simulink subsystem "Shooter_Controls_sub"  (R2023b)
settings: Solver=VariableStepAuto  StartTime=0.0  StopTime=10.0  RelTol=1e-3
undefined symbols (not defined in the file): Feeder_Max_Pulsetime, Field_BlueAllianceZoneX, Field_RedAllianceZoneX, Rebuilt_Feeder_Motor_Gain_FF, Rebuilt_Feeder_Time_FWD, Rebuilt_Feeder_Time_REV, Rebuilt_Hood_Servo_Pos_Min, Rebuilt_Match_Time_Auto_Timer, Rebuilt_Match_Time_End_Game_Timer, Rebuilt_Match_Time_Shift_1, Rebuilt_Match_Time_Shift_2, Rebuilt_Match_Time_Shift_3, Rebuilt_Match_Time_Shift_4, Rebuilt_Match_Time_Shift_Timer, Rebuilt_Match_Time_Shoot_Early, Rebuilt_Match_Time_Transition, Rebuilt_Negative_Feeder_Speed, Rebuilt_Shoot_Hood_Pos_Max_Error, Rebuilt_Shoot_Motor_Max_Error, Rebuilt_Shoot_Robot_Velocity_Max, Rebuilt_Shooter_Error_Integral_Enable, Rebuilt_Shooter_Motor_Gain_FF, Rebuilt_Shooter_Motor_Gain_I, Rebuilt_Shooter_Motor_Gain_I_Low, Rebuilt_Shooter_Motor_Gain_P, Rebuilt_Target_Feeder_Speed, Rebuilt_Target_Transfer_Speed, Rebuilt_Transfer_Error_Integral_Enable, Rebuilt_Transfer_Minimum_Factor, t_sample
libraries: simulink x20, Controls_Components_lib x2
(part 1 of 2)
settings Model: Creator=ander  LastModifiedBy=FIRSTMentor

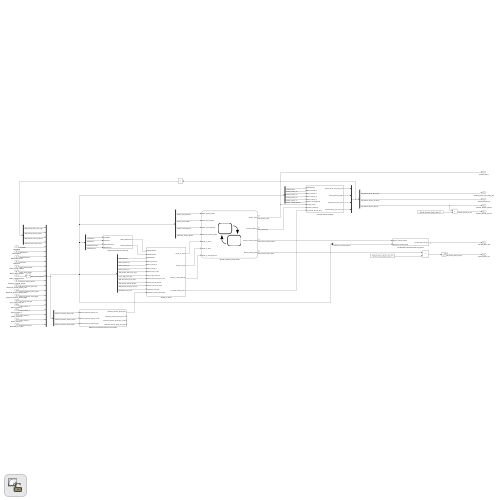
[thumbnail: Simulink's stored preview of the top-level diagram]
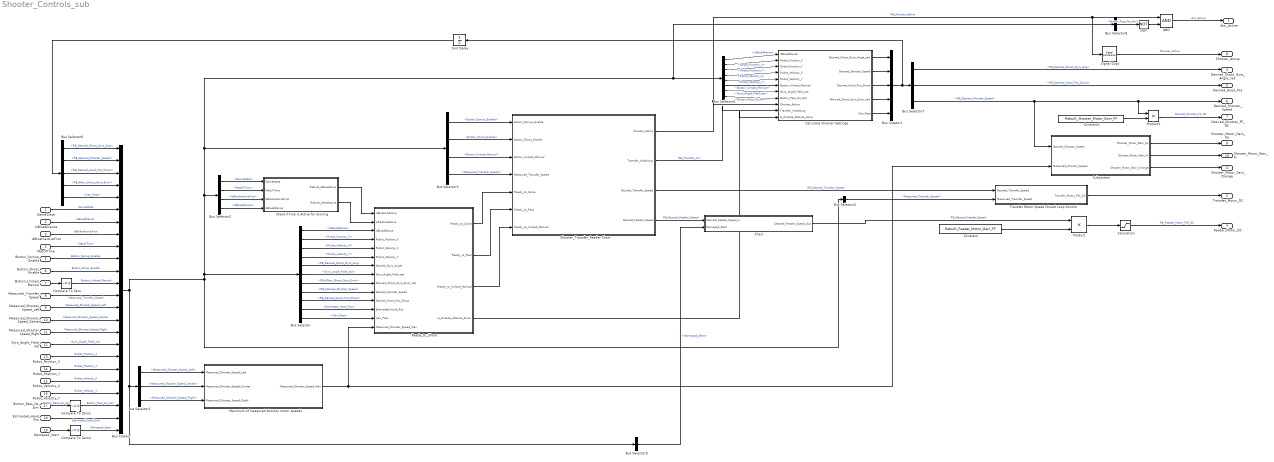
== system Shooter_Controls_sub ==
  GameState : Inport
  IsBlueAlliance : Inport  Port=2
  IsBlueInactiveFirst : Inport  Port=3
  MatchTime : Inport  Port=4
  Button_Spinup_Enable : Inport  Port=5
  Button_Shoot_Enable : Inport  Port=6
  Button_Unload_Manual : Inport  Port=7
  Measured_Transfer_Speed : Inport  Port=8
  Measured_Shooter_Speed_Left : Inport  Port=9
  Measured_Shooter_Speed_Center : Inport  Port=10
  Measured_Shooter_Speed_Right : Inport  Port=11
  Gyro_Angle_Field_rad : Inport  Port=12
  Robot_Position_X : Inport  Port=13
  Robot_Position_Y : Inport  Port=14
  Robot_Velocity_X : Inport  Port=15
  Robot_Velocity_Y : Inport  Port=16
  Button_Pass_No_Aim : Inport  Port=17
  Gamepad_Start : Inport  Port=18
  Estimated_Hood_Pos : Inport  Port=19
  AND : Logic  AllPortsSameDT=off  OutDataTypeStr=boolean
  Bus Creator : BusCreator  Inputs=24
  Bus Selector : BusSelector  OutputSignals=IsBlueAlliance,Robot_Position_X,Robot_Velocity_X,Robot_Velocity_Y,RB_Desired_Shoot_Gyro_Ang,Gyro_Angle_Field_rad,RB_Allow_Shoot_Gyro_Error,RB_Desired_Shooter_Speed,RB_Desired_Hood_Pos_Shoot,Estimated_Hood_Pos,Can_Pass
  Bus Selector1 : BusSelector  OutputSignals=Measured_Shooter_Speed_Left,Measured_Shooter_Speed_Center,Measured_Shooter_Speed_Right
  Bus Selector2 : BusSelector  OutputSignals=GameState,MatchTime,IsBlueInactiveFirst,IsBlueAlliance
  Bus Selector3 : BusSelector  OutputSignals=Button_Spinup_Enable,Button_Shoot_Enable,Button_Unload_Manual,Measured_Transfer_Speed
  Bus Selector4 : BusSelector  OutputSignals=Measured_Transfer_Speed
  Bus Selector5 : BusSelector  OutputSignals=IsBlueAlliance,Robot_Position_X,Robot_Position_Y,Robot_Velocity_X,Robot_Velocity_Y,Button_Unload_Manual,Gyro_Angle_Field_rad,Button_Pass_No_Aim
  Bus Selector6 : BusSelector  OutputSignals=RB_Desired_Shoot_Gyro_Ang,RB_Desired_Shooter_Speed,RB_Desired_Hood_Pos_Shoot,RB_Allow_Shoot_Gyro_Error,Can_Pass
  Bus Selector7 : BusSelector  OutputSignals=RB_Desired_Shoot_Gyro_Ang,RB_Desired_Hood_Pos_Shoot,RB_Desired_Shooter_Speed
  Bus Selector8 : BusSelector  OutputSignals=Button_Pass_No_Aim
  Bus Selector9 : BusSelector  OutputSignals=Gamepad_Start
  Bus Creator1 : BusCreator  Inputs=5
  Calculate Shooter Settings : Subsystem
  Chart : Stateflow chart  TreatAsAtomicUnit=on
  Check if Hub is Active for Scoring : Subsystem
  Compare To Zero : simulink/Logic and Bit Operations/Compare To Zero  relop=~=  OutDataTypeStr=boolean
  Compare To Zero1 : simulink/Logic and Bit Operations/Compare To Zero  relop=~=  OutDataTypeStr=boolean
  Compare To Zero2 : simulink/Logic and Bit Operations/Compare To Zero  relop=~=  OutDataTypeStr=boolean
  Constant : Constant  Value=Rebuilt_Feeder_Motor_Gain_FF
  Constant1 : Constant  Value=Rebuilt_Shooter_Motor_Gain_FF
  Maximum of measured shooter motor speeds : Subsystem
  NOT : Logic  Operator=NOT  AllPortsSameDT=off  OutDataTypeStr=boolean
  Product : Product
  Product1 : Product
  Ready_to_Shoot : Subsystem
  Saturation : Saturate  UpperLimit=1  LowerLimit=-1
  Shooter_Transfer_Feeder Chart : Stateflow chart  TreatAsAtomicUnit=on
      settings: PortSchema="{\"entries\":[{\"content\":{\"sides\":[{\"content\":{\"connectorIds\":[\"In3\",\"In4\",\"In5\",\"In1\",\"In2\",\"In6\",\"In7\"]},\"type\":\"ConnectorPlacement.EquallySpacedRectSide\",\"uuid\":\"74f441ca-e68c-42da-ab23-bb4c7b61ec4f\"},{\"content\":{\"connectorIds\":[\"Out1\",\"Out4\",\"Out3\",\"Out2\"],\"side\":\"RIGHT\"},\"type\":\"ConnectorPlacement.EquallySpacedRectSide\",\"uuid\":\"2fadc481-2bc8-4130-a1bd-49ae230fca41\"},{\"content\":{\"side\":\"TOP\"},\"type\":\"ConnectorPlacement.EquallySpacedRectSide\",\"uuid\":\"2ae77c41-2153-497e-bbb0-d4cfaeee089b\"}]},\"type\":\"ConnectorPlacement.EquallySpacedConnector\",\"uuid\":\"7b036f05-bc25-4046-a317-cc0a6fa71ced\"}],\"packageUris\":[\"http://schema.mathworks.com/mf0/Connector/R2020b\"],\"version\":\"1.0\"}"
  Signal Copy : SignalConversion  OverrideOpt=off
  Subsystem : Subsystem
  Transfer Motor Speed Closed Loop Control : Subsystem
  Unit Delay : UnitDelay  SampleTime=-1  HasFrameUpgradeWarning=on
  Aim_Active : Outport
  Transfer_Motor_DC : Outport  Port=2
  Feeder_Motor_DC : Outport  Port=3
  Desired_Shoot_Gyro_Angle_rad : Outport  Port=4
  Desired_Hood_Pos : Outport  Port=5
  Desired_Shooter_Speed : Outport  Port=6
  Desired_Shooter_FF_DC : Outport  Port=7
  Shooter_Active : Outport  Port=8
  Shooter_Motor_Gain_Kp : Outport  Port=9
  Shooter_Motor_Gain_Ki : Outport  Port=10
  Shooter_Motor_Gain_Change : Outport  Port=11
  wires:
  Shooter_Transfer_Feeder Chart/1(Shooter_Active) -> Calculate Shooter Settings/9(Shooter_Active), Signal Copy/1, AND/1  "RB_Shooter_Active"
  Check if Hub is Active for Scoring/1(Rebuilt_IsBlueActive) -> Ready_to_Shoot/1(isBlueHubActive)
  Check if Hub is Active for Scoring/2(Rebuilt_IsRedActive) -> Ready_to_Shoot/2(isRedHubActive)
  Ready_to_Shoot/1(Ready_to_Score) -> Shooter_Transfer_Feeder Chart/2(Ready_to_Score)
  Bus Creator/1 -> Bus Selector1/1, Bus Selector9/1, Bus Selector4/1, Bus Selector2/1, Bus Selector3/1, Bus Selector5/1, Bus Selector8/1, Bus Selector/1
  Bus Selector/6 -> Ready_to_Shoot/8(Gyro_Angle_Field_rad)  "<Gyro_Angle_Field_rad>"
  Bus Selector/5 -> Ready_to_Shoot/7(Desired_Gyro_Angle)  "<RB_Desired_Shoot_Gyro_Ang>"
  Bus Selector/8 -> Ready_to_Shoot/10(Desired_Shooter_Speed)  "<RB_Desired_Shooter_Speed>"
  Bus Selector/2 -> Ready_to_Shoot/4(Robot_Position_X)  "<Robot_Position_X>"
  Bus Selector/1 -> Ready_to_Shoot/3(isBlueAlliance)  "<IsBlueAlliance>"
  Bus Selector2/2 -> Check if Hub is Active for Scoring/2(MatchTime)  "<MatchTime>"
  Bus Selector2/3 -> Check if Hub is Active for Scoring/3(IsBlueInactiveFirst)  "<IsBlueInactiveFirst>"
  Bus Selector3/1 -> Shooter_Transfer_Feeder Chart/3(Button_Spinup_Enable)  "<Button_Spinup_Enable>"
  Bus Selector3/2 -> Shooter_Transfer_Feeder Chart/4(Button_Shoot_Enable)  "<Button_Shoot_Enable>"
  Bus Selector3/4 -> Shooter_Transfer_Feeder Chart/1(Measured_Transfer_Speed)  "<Measured_Transfer_Speed>"
  Product/1 -> Saturation/1
  Shooter_Transfer_Feeder Chart/3(Desired_Transfer_Speed) -> Transfer Motor Speed Closed Loop Control/1(Desired_Transfer_Speed)  "RB_Desired_Transfer_Speed"
  Bus Selector4/1 -> Transfer Motor Speed Closed Loop Control/2(Measured_Transfer_Speed)  "<Measured_Transfer_Speed>"
  Transfer Motor Speed Closed Loop Control/1(Transfer_Motor_PID_DC) -> Transfer_Motor_DC/1
  Bus Selector5/2 -> Calculate Shooter Settings/2(Robot_Position_X)  "<Robot_Position_X>"
  Bus Selector5/3 -> Calculate Shooter Settings/3(Robot_Position_Y)  "<Robot_Position_Y>"
  Calculate Shooter Settings/1(Desired_Shoot_Gyro_Angle_rad) -> Bus Creator1/1
  Calculate Shooter Settings/2(Desired_Shooter_Speed) -> Bus Creator1/2
  Calculate Shooter Settings/3(Desired_Hood_Pos_Shoot) -> Bus Creator1/3
  Bus Creator1/1 -> Bus Selector7/1, Unit Delay/1
  Unit Delay/1 -> Bus Selector6/1
  Bus Selector5/1 -> Calculate Shooter Settings/1(IsBlueAlliance)  "<IsBlueAlliance>"
  Constant/1 -> Product/2
  Bus Selector6/1 -> Bus Creator/1  "<RB_Desired_Shoot_Gyro_Ang>"
  Bus Selector6/2 -> Bus Creator/2  "<RB_Desired_Shooter_Speed>"
  Bus Selector6/3 -> Bus Creator/3  "<RB_Desired_Hood_Pos_Shoot>"
  Gyro_Angle_Field_rad/1 -> Bus Creator/17  "Gyro_Angle_Field_rad"
  Robot_Position_X/1 -> Bus Creator/18  "Robot_Position_X"
  Robot_Position_Y/1 -> Bus Creator/19  "Robot_Position_Y"
  Robot_Velocity_X/1 -> Bus Creator/20  "Robot_Velocity_X"
  Robot_Velocity_Y/1 -> Bus Creator/21  "Robot_Velocity_Y"
  Bus Selector5/4 -> Calculate Shooter Settings/4(Robot_Velocity_X)  "<Robot_Velocity_X>"
  Bus Selector5/5 -> Calculate Shooter Settings/5(Robot_Velocity_Y)  "<Robot_Velocity_Y>"
  Bus Selector7/1 -> Desired_Shoot_Gyro_Angle_rad/1  "<RB_Desired_Shoot_Gyro_Ang>"
  Bus Selector7/2 -> Desired_Hood_Pos/1  "<RB_Desired_Hood_Pos_Shoot>"
  Bus Selector7/3 -> Desired_Shooter_Speed/1, Product1/1, Subsystem/1(Desired_Shooter_Speed)  "<RB_Desired_Shooter_Speed>"
  Ready_to_Shoot/2(Ready_to_Pass) -> Shooter_Transfer_Feeder Chart/6(Ready_to_Pass)
  Ready_to_Shoot/4(Is_Outside_Alliance_Zone) -> Calculate Shooter Settings/11(Is_Outside_Alliance_Zone)
  Bus Selector2/1 -> Check if Hub is Active for Scoring/1(GameState)  "<GameState>"
  GameState/1 -> Bus Creator/6  "GameState"
  IsBlueAlliance/1 -> Bus Creator/7  "IsBlueAlliance"
  IsBlueInactiveFirst/1 -> Bus Creator/8  "IsBlueInactiveFirst"
  MatchTime/1 -> Bus Creator/9  "MatchTime"
  Button_Spinup_Enable/1 -> Bus Creator/10  "Button_Spinup_Enable"
  Button_Shoot_Enable/1 -> Bus Creator/11  "Button_Shoot_Enable"
  Measured_Transfer_Speed/1 -> Bus Creator/13  "Measured_Transfer_Speed"
  Measured_Shooter_Speed_Left/1 -> Bus Creator/14  "Measured_Shooter_Speed_Left"
  Measured_Shooter_Speed_Center/1 -> Bus Creator/15  "Measured_Shooter_Speed_Center"
  Measured_Shooter_Speed_Right/1 -> Bus Creator/16  "Measured_Shooter_Speed_Right"
  Calculate Shooter Settings/4(Allowed_Shoot_Gyro_Error_rad) -> Bus Creator1/4
  Bus Selector6/4 -> Bus Creator/4  "<RB_Allow_Shoot_Gyro_Error>"
  Bus Selector/3 -> Ready_to_Shoot/5(Robot_Velocity_X)  "<Robot_Velocity_X>"
  Bus Selector/4 -> Ready_to_Shoot/6(Robot_Velocity_Y)  "<Robot_Velocity_Y>"
  Bus Selector/7 -> Ready_to_Shoot/9(Allowed_Shoot_Gyro_Error_rad)  "<RB_Allow_Shoot_Gyro_Error>"
  Bus Selector/9 -> Ready_to_Shoot/11(Desired_Hood_Pos_Shoot)  "<RB_Desired_Hood_Pos_Shoot>"
  Bus Selector1/1 -> Maximum of measured shooter motor speeds/1(Measured_Shooter_Speed_Left)  "<Measured_Shooter_Speed_Left>"
  Bus Selector1/2 -> Maximum of measured shooter motor speeds/2(Measured_Shooter_Speed_Center)  "<Measured_Shooter_Speed_Center>"
  Bus Selector1/3 -> Maximum of measured shooter motor speeds/3(Measured_Shooter_Speed_Right)  "<Measured_Shooter_Speed_Right>"
  Bus Selector/10 -> Ready_to_Shoot/12(Estimated_Hood_Pos)  "<Estimated_Hood_Pos>"
  Shooter_Transfer_Feeder Chart/4(Transfer_Initializing) -> Calculate Shooter Settings/10(Transfer_Initializing)  "RB_Transfer_Init"
  Saturation/1 -> Feeder_Motor_DC/1  "RB_Feeder_Motor_PID_DC"
  Bus Selector2/4 -> Check if Hub is Active for Scoring/4(IsBlueAlliance)  "<IsBlueAlliance>"
  Ready_to_Shoot/3(Ready_to_Unload_Manual) -> Shooter_Transfer_Feeder Chart/7(Ready_to_Unload_Manual)
  Button_Unload_Manual/1 -> Compare To Zero/1
  Bus Selector3/3 -> Shooter_Transfer_Feeder Chart/5(Button_Unload_Manual)  "<Button_Unload_Manual>"
  Bus Selector5/6 -> Calculate Shooter Settings/6(Button_Unload_Manual)  "<Button_Unload_Manual>"
  Compare To Zero/1 -> Bus Creator/12  "Button_Unload_Manual"
  Product1/1 -> Desired_Shooter_FF_DC/1  "Desired_Shooter_FF_DC"
  Constant1/1 -> Product1/2
  Bus Selector5/7 -> Calculate Shooter Settings/7(Gyro_Angle_Field_rad)  "<Gyro_Angle_Field_rad>"
  Bus Selector5/8 -> Calculate Shooter Settings/8(Button_Pass_No_Aim)  "<Button_Pass_No_Aim>"
  AND/1 -> Aim_Active/1  "Aim_Active"
  Calculate Shooter Settings/5(Can_Pass) -> Bus Creator1/5
  Bus Selector8/1 -> NOT/1  "<Button_Pass_No_Aim>"
  Signal Copy/1 -> Shooter_Active/1  "Shooter_Active"
  Bus Selector6/5 -> Bus Creator/5  "<Can_Pass>"
  Estimated_Hood_Pos/1 -> Bus Creator/23  "Estimated_Hood_Pos"
  Button_Pass_No_Aim/1 -> Compare To Zero1/1  "Button_Pass_No_Aim"
  Bus Selector/11 -> Ready_to_Shoot/13(Can_Pass)  "<Can_Pass>"
  NOT/1 -> AND/2
  Compare To Zero1/1 -> Bus Creator/22  "Button_Pass_No_Aim"
  Maximum of measured shooter motor speeds/1(Measured_Shooter_Speed_Max) -> Ready_to_Shoot/14(Measured_Shooter_Speed_Max), Subsystem/2(Measured_Shooter_Speed)
  Subsystem/1(Shooter_Motor_Gain_Kp) -> Shooter_Motor_Gain_Kp/1
  Subsystem/2(Shooter_Motor_Gain_Ki) -> Shooter_Motor_Gain_Ki/1
  Subsystem/3(Shooter_Motor_Gain_Change) -> Shooter_Motor_Gain_Change/1
  Gamepad_Start/1 -> Compare To Zero2/1
  Bus Selector9/1 -> Chart/2(Gamepad_Start)  "<Gamepad_Start>"
  Shooter_Transfer_Feeder Chart/2(Desired_Feeder_Speed) -> Chart/1(Desired_Feeder_Speed_In)  "RB_Desired_Feeder_Speed"
  Chart/1(Desired_Feeder_Speed_Out) -> Product/1  "RB_Desired_Feeder_Speed"
  Compare To Zero2/1 -> Bus Creator/24  "Gamepad_Start"

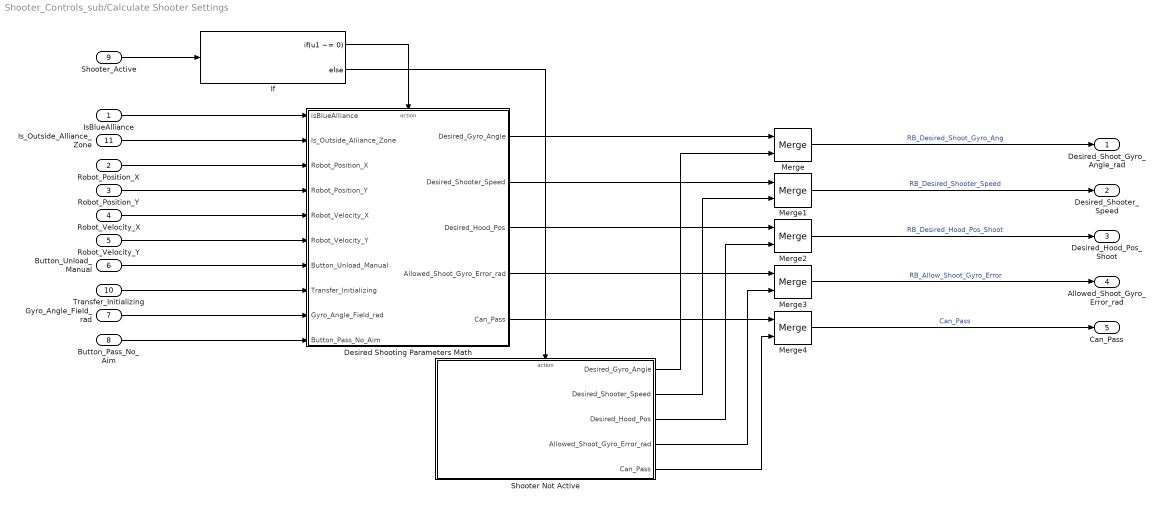
== system Shooter_Controls_sub/Calculate Shooter Settings ==
  IsBlueAlliance : Inport
  Robot_Position_X : Inport  Port=2
  Robot_Position_Y : Inport  Port=3
  Robot_Velocity_X : Inport  Port=4
  Robot_Velocity_Y : Inport  Port=5
  Button_Unload_Manual : Inport  Port=6
  Gyro_Angle_Field_rad : Inport  Port=7
  Button_Pass_No_Aim : Inport  Port=8
  Shooter_Active : Inport  Port=9
  Transfer_Initializing : Inport  Port=10
  Is_Outside_Alliance_Zone : Inport  Port=11
  Desired Shooting Parameters Math : Subsystem
  If : If  IfExpression=u1 ~= 0
  Merge{,1..4} (5 alike) : Merge
  Shooter Not Active : Subsystem
  Desired_Shoot_Gyro_Angle_rad : Outport
  Desired_Shooter_Speed : Outport  Port=2
  Desired_Hood_Pos_Shoot : Outport  Port=3
  Allowed_Shoot_Gyro_Error_rad : Outport  Port=4
  Can_Pass : Outport  Port=5
  wires:
  Merge4/1 -> Can_Pass/1  "Can_Pass"
  Shooter Not Active/5(Can_Pass) -> Merge4/2
  Desired Shooting Parameters Math/5(Can_Pass) -> Merge4/1
  Button_Pass_No_Aim/1 -> Desired Shooting Parameters Math/10(Button_Pass_No_Aim)
  Gyro_Angle_Field_rad/1 -> Desired Shooting Parameters Math/9(Gyro_Angle_Field_rad)
  Button_Unload_Manual/1 -> Desired Shooting Parameters Math/7(Button_Unload_Manual)
  Transfer_Initializing/1 -> Desired Shooting Parameters Math/8(Transfer_Initializing)
  Is_Outside_Alliance_Zone/1 -> Desired Shooting Parameters Math/2(Is_Outside_Alliance_Zone)
  Shooter Not Active/4(Allowed_Shoot_Gyro_Error_rad) -> Merge3/2
  Shooter Not Active/3(Desired_Hood_Pos) -> Merge2/2
  Shooter Not Active/2(Desired_Shooter_Speed) -> Merge1/2
  Shooter Not Active/1(Desired_Gyro_Angle) -> Merge/2
  Desired Shooting Parameters Math/4(Allowed_Shoot_Gyro_Error_rad) -> Merge3/1
  Desired Shooting Parameters Math/3(Desired_Hood_Pos) -> Merge2/1
  Desired Shooting Parameters Math/2(Desired_Shooter_Speed) -> Merge1/1
  Desired Shooting Parameters Math/1(Desired_Gyro_Angle) -> Merge/1
  Robot_Velocity_Y/1 -> Desired Shooting Parameters Math/6(Robot_Velocity_Y)
  Robot_Velocity_X/1 -> Desired Shooting Parameters Math/5(Robot_Velocity_X)
  Robot_Position_Y/1 -> Desired Shooting Parameters Math/4(Robot_Position_Y)
  Robot_Position_X/1 -> Desired Shooting Parameters Math/3(Robot_Position_X)
  IsBlueAlliance/1 -> Desired Shooting Parameters Math/1(isBlueAlliance)
  Merge3/1 -> Allowed_Shoot_Gyro_Error_rad/1  "RB_Allow_Shoot_Gyro_Error"
  If/2 -> Shooter Not Active/Action
  Shooter_Active/1 -> If/1
  Merge1/1 -> Desired_Shooter_Speed/1  "RB_Desired_Shooter_Speed"
  If/1 -> Desired Shooting Parameters Math/Action
  Merge/1 -> Desired_Shoot_Gyro_Angle_rad/1  "RB_Desired_Shoot_Gyro_Ang"
  Merge2/1 -> Desired_Hood_Pos_Shoot/1  "RB_Desired_Hood_Pos_Shoot"

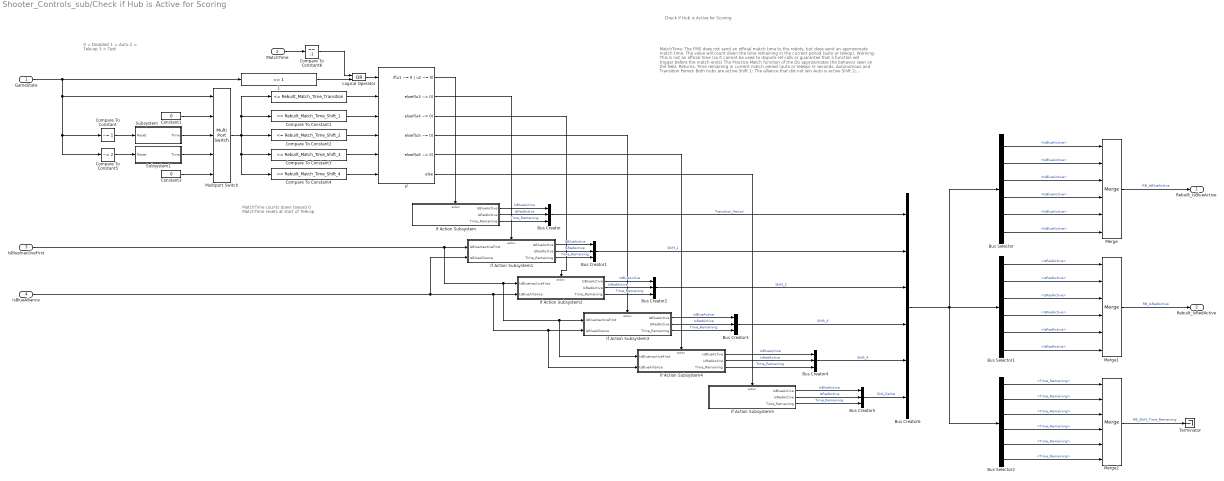
== system Shooter_Controls_sub/Check if Hub is Active for Scoring ==
  note: MatchTime counts down toward 0
      | MatchTime resets at start of Tele-op
  note: Check if Hub is Active for Scoring
  note: MatchTime: The FMS does not send an official match time to the robots, but does send an approximate match time. The value will count down the time remaining in the current period (auto or teleop). Warning: This is not an official time (so it cannot be used to dispute ref calls or guarantee that a function will trigger before the match ends) The Practice Match function of the DS approximates the behavior seen on the field.
      | Returns: Time remaining in current match period (auto or teleop) in seconds.
      |
      | Autonomous and Transition Period: Both hubs are active
      | Shift 1: The alliance that did not win Auto is active
      | Shift 2: Opposite of Shift 1
      | Shift 3: Same as Shift 1
      | Shift 4: Same as Shift 2
      | Endgame: Both hubs are active
  note: 0 = Disabled
      | 1 = Auto
      | 2 = Tele-op
      | 3 = Test
  GameState : Inport
  MatchTime : Inport  Port=2
  IsBlueInactiveFirst : Inport  Port=3
  IsBlueAlliance : Inport  Port=4
  " " : simulink/Logic and Bit Operations/Compare To Constant  relop=<=  const=Rebuilt_Match_Time_Transition  OutDataTypeStr=boolean
  " 1" : simulink/Logic and Bit Operations/Compare To Constant  relop===  const=1  OutDataTypeStr=boolean
  Bus Creator{,1..5} (6 alike) : BusCreator  Inputs=3
  Bus Creator6 : BusCreator  Inputs=6
  Bus Selector : BusSelector  OutputSignals=Transition_Period.IsBlueActive,Shift_1.IsBlueActive,Shift_2.IsBlueActive,Shift_3.IsBlueActive,Shift_4.IsBlueActive,End_Game.IsBlueActive
  Bus Selector1 : BusSelector  OutputSignals=Transition_Period.IsRedActive,Shift_1.IsRedActive,Shift_2.IsRedActive,Shift_3.IsRedActive,Shift_4.IsRedActive,End_Game.IsRedActive
  Bus Selector2 : BusSelector  OutputSignals=Transition_Period.Time_Remaining,Shift_1.Time_Remaining,Shift_2.Time_Remaining,Shift_3.Time_Remaining,Shift_4.Time_Remaining,End_Game.Time_Remaining
  Compare To Constant : simulink/Logic and Bit Operations/Compare To Constant  relop=~=  const=1  OutDataTypeStr=boolean
  Compare To Constant1 : simulink/Logic and Bit Operations/Compare To Constant  relop=<=  const=Rebuilt_Match_Time_Shift_1  OutDataTypeStr=boolean
  Compare To Constant2 : simulink/Logic and Bit Operations/Compare To Constant  relop=<=  const=Rebuilt_Match_Time_Shift_2  OutDataTypeStr=boolean
  Compare To Constant3 : simulink/Logic and Bit Operations/Compare To Constant  relop=<=  const=Rebuilt_Match_Time_Shift_3  OutDataTypeStr=boolean
  Compare To Constant4 : simulink/Logic and Bit Operations/Compare To Constant  relop=<=  const=Rebuilt_Match_Time_Shift_4  OutDataTypeStr=boolean
  Compare To Constant5 : simulink/Logic and Bit Operations/Compare To Constant  relop=~=  const=2  OutDataTypeStr=boolean
  Compare To Constant6 : simulink/Logic and Bit Operations/Compare To Constant  relop===  const=-1  OutDataTypeStr=boolean
  Constant1 : Constant  Value=0
  Constant3 : Constant  Value=0
  If : If  NumInputs=6  IfExpression=u1 ~= 0 | u2 ~= 0  ElseIfExpressions=u3 ~= 0,u4 ~= 0,u5 ~= 0,u6 ~= 0
  If Action Subsystem : Subsystem  TreatAsAtomicUnit=on
  If Action Subsystem1 : Subsystem  TreatAsAtomicUnit=on
  If Action Subsystem2 : Subsystem  TreatAsAtomicUnit=on
  If Action Subsystem3 : Subsystem  TreatAsAtomicUnit=on
  If Action Subsystem4 : Subsystem  TreatAsAtomicUnit=on
  If Action Subsystem5 : Subsystem  TreatAsAtomicUnit=on
  Logical Operator : Logic  Operator=OR  AllPortsSameDT=off  OutDataTypeStr=boolean
  Merge : Merge  Inputs=6
  Merge1 : Merge  Inputs=6
  Merge2 : Merge  Inputs=6
  Multiport Switch : MultiPortSwitch  DataPortOrder=Zero-based contiguous  Inputs=4  zeroidx=on  SaturateOnIntegerOverflow=off  InputSameDT=off
  Subsystem : Subsystem
  Subsystem1 : Subsystem
  Terminator : Terminator
  Rebuilt_IsBlueActive : Outport
  Rebuilt_IsRedActive : Outport  Port=2
  wires:
  Compare To Constant6/1 -> Logical Operator/1
  Logical Operator/1 -> If/1
  " 1"/1 -> Logical Operator/2
  MatchTime/1 -> Compare To Constant6/1
  Compare To Constant5/1 -> Subsystem1/1(Reset)
  Subsystem1/1(Time) -> Multiport Switch/4
  Compare To Constant/1 -> Subsystem/1(Reset)
  Subsystem/1(Time) -> Multiport Switch/3
  Constant3/1 -> Multiport Switch/5
  Constant1/1 -> Multiport Switch/2
  Multiport Switch/1 -> " "/1, Compare To Constant1/1, Compare To Constant4/1, Compare To Constant3/1, Compare To Constant2/1
  IsBlueAlliance/1 -> If Action Subsystem2/2(IsBlueAlliance), If Action Subsystem3/2(IsBlueAlliance), If Action Subsystem4/2(IsBlueAlliance), If Action Subsystem1/2(IsBlueAlliance)
  GameState/1 -> Multiport Switch/1, Compare To Constant/1, Compare To Constant5/1, " 1"/1
  Compare To Constant4/1 -> If/6
  Compare To Constant3/1 -> If/5
  Compare To Constant2/1 -> If/4
  Compare To Constant1/1 -> If/3
  " "/1 -> If/2
  If Action Subsystem5/3(Time_Remaining) -> Bus Creator5/3  "Time_Remaining"
  If Action Subsystem4/3(Time_Remaining) -> Bus Creator4/3  "Time_Remaining"
  If Action Subsystem3/3(Time_Remaining) -> Bus Creator3/3  "Time_Remaining"
  If Action Subsystem2/3(Time_Remaining) -> Bus Creator2/3  "Time_Remaining"
  Merge2/1 -> Terminator/1  "RB_Shift_Time_Remaining"
  Bus Selector2/6 -> Merge2/6  "<Time_Remaining>"
  Bus Selector2/5 -> Merge2/5  "<Time_Remaining>"
  Bus Selector2/4 -> Merge2/4  "<Time_Remaining>"
  Bus Selector2/3 -> Merge2/3  "<Time_Remaining>"
  Bus Selector2/2 -> Merge2/2  "<Time_Remaining>"
  Bus Selector2/1 -> Merge2/1  "<Time_Remaining>"
  Bus Selector1/6 -> Merge1/6  "<IsRedActive>"
  Bus Selector1/5 -> Merge1/5  "<IsRedActive>"
  Bus Selector1/4 -> Merge1/4  "<IsRedActive>"
  Bus Selector1/3 -> Merge1/3  "<IsRedActive>"
  Bus Selector1/2 -> Merge1/2  "<IsRedActive>"
  Bus Selector1/1 -> Merge1/1  "<IsRedActive>"
  Bus Selector/6 -> Merge/6  "<IsBlueActive>"
  Bus Selector/5 -> Merge/5  "<IsBlueActive>"
  Bus Selector/4 -> Merge/4  "<IsBlueActive>"
  Bus Selector/3 -> Merge/3  "<IsBlueActive>"
  Bus Selector/2 -> Merge/2  "<IsBlueActive>"
  Bus Selector/1 -> Merge/1  "<IsBlueActive>"
  Bus Creator6/1 -> Bus Selector2/1, Bus Selector1/1, Bus Selector/1
  Bus Creator5/1 -> Bus Creator6/6  "End_Game"
  Bus Creator4/1 -> Bus Creator6/5  "Shift_4"
  Bus Creator3/1 -> Bus Creator6/4  "Shift_3"
  Bus Creator2/1 -> Bus Creator6/3  "Shift_2"
  Bus Creator1/1 -> Bus Creator6/2  "Shift_1"
  Bus Creator/1 -> Bus Creator6/1  "Transition_Period"
  If Action Subsystem5/2(IsRedActive) -> Bus Creator5/2  "IsRedActive"
  If Action Subsystem5/1(IsBlueActive) -> Bus Creator5/1  "IsBlueActive"
  If Action Subsystem4/2(IsRedActive) -> Bus Creator4/2  "IsRedActive"
  If Action Subsystem4/1(IsBlueActive) -> Bus Creator4/1  "IsBlueActive"
  If Action Subsystem3/2(IsRedActive) -> Bus Creator3/2  "IsRedActive"
  If Action Subsystem3/1(IsBlueActive) -> Bus Creator3/1  "IsBlueActive"
  If Action Subsystem2/2(IsRedActive) -> Bus Creator2/2  "IsRedActive"
  If Action Subsystem2/1(IsBlueActive) -> Bus Creator2/1  "IsBlueActive"
  If Action Subsystem1/3(Time_Remaining) -> Bus Creator1/3  "Time_Remaining"
  If Action Subsystem1/2(IsRedActive) -> Bus Creator1/2  "IsRedActive"
  If Action Subsystem1/1(IsBlueActive) -> Bus Creator1/1  "IsBlueActive"
  If Action Subsystem/3(Time_Remaining) -> Bus Creator/3  "Time_Remaining"
  If Action Subsystem/2(IsRedActive) -> Bus Creator/2  "IsRedActive"
  If Action Subsystem/1(IsBlueActive) -> Bus Creator/1  "IsBlueActive"
  Merge1/1 -> Rebuilt_IsRedActive/1  "RB_IsRedActive"
  Merge/1 -> Rebuilt_IsBlueActive/1  "RB_IsBlueActive"
  If/6 -> If Action Subsystem5/Action
  If/5 -> If Action Subsystem4/Action
  If/4 -> If Action Subsystem3/Action
  If/3 -> If Action Subsystem2/Action
  If/2 -> If Action Subsystem1/Action
  IsBlueInactiveFirst/1 -> If Action Subsystem1/1(IsBlueInactiveFirst), If Action Subsystem2/1(IsBlueInactiveFirst), If Action Subsystem3/1(IsBlueInactiveFirst), If Action Subsystem4/1(IsBlueInactiveFirst)
  If/1 -> If Action Subsystem/Action

== system Shooter_Controls_sub/Maximum of measured shooter motor speeds ==
  note: The three sets of shooter wheels are all connected together on a single hex shaft.
      |
      | Three motors are connected to the single hex shaft through independent belts and pulleys.
      |
      | Each of the motors are running close to the same speed, but not exactly due to the slight differences in pulleys and flex in the belts.
      |
      | Take the absolute value of each motor speed (mounting differences will cause some to be positive and others negative) and then take the maximum of the three. This allows the robot to keep working if one motor fails.
  note: Calculate Measured Shooter Motor Speed Maximum
  Measured_Shooter_Speed_Left : Inport
  Measured_Shooter_Speed_Center : Inport  Port=2
  Measured_Shooter_Speed_Right : Inport  Port=3
  Abs1 : Abs  SaturateOnIntegerOverflow=off
  Abs2 : Abs  SaturateOnIntegerOverflow=off
  Abs3 : Abs  SaturateOnIntegerOverflow=off
  Max : MinMax  Function=max  Inputs=3
  Measured_Shooter_Speed_Max : Outport
  wires:
  Abs2/1 -> Max/1
  Max/1 -> Measured_Shooter_Speed_Max/1  "RB_Meas_Shooter_Speed_Max"
  Abs3/1 -> Max/3
  Abs1/1 -> Max/2
  Measured_Shooter_Speed_Right/1 -> Abs3/1  "Measured_Shooter_Speed_Right"
  Measured_Shooter_Speed_Center/1 -> Abs1/1  "Measured_Shooter_Speed_Center"
  Measured_Shooter_Speed_Left/1 -> Abs2/1  "Measured_Shooter_Speed_Left"

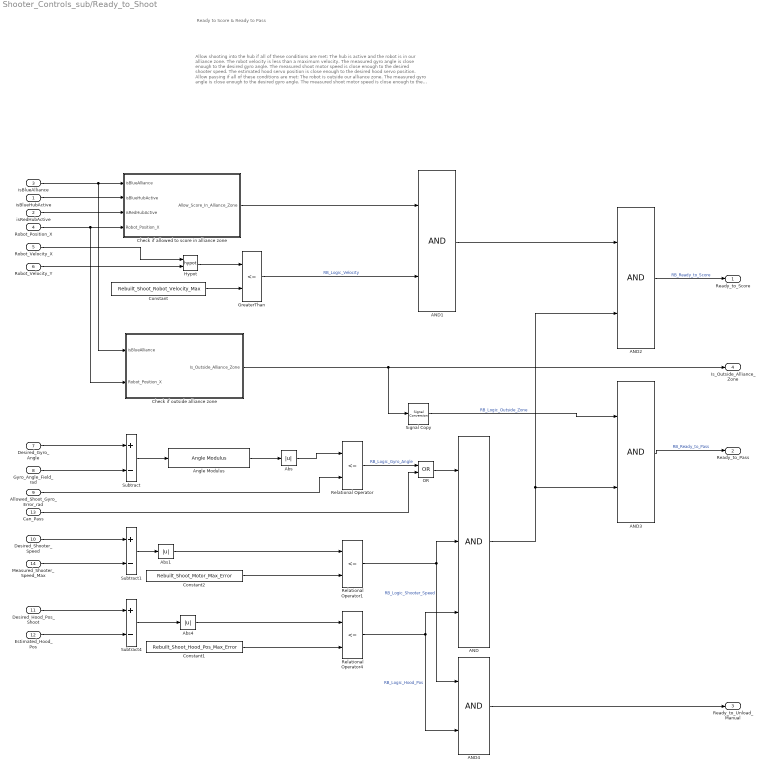
== system Shooter_Controls_sub/Ready_to_Shoot ==
  note: Allow shooting into the hub if all of these conditions are met:
      | The hub is active and the robot is in our alliance zone.
      | The robot velocity is less than a maximum velocity.
      | The measured gyro angle is close enough to the desired gyro angle.
      | The measured shoot motor speed is close enough to the desired shooter speed.
      | The estimated hood servo position is close enough to the desired hood servo position.
      |
      | Allow passing if all of these conditions are met:
      | The robot is outside our alliance zone.
      | The measured gyro angle is close enough to the desired gyro angle.
      | The measured shoot motor speed is close enough to the desired shooter speed. Do this for 3 motors.
      | The estimated hood servo position is close enough to the desired hood servo position.
  note: Ready to Score & Ready to Pass
  isBlueHubActive : Inport
  isRedHubActive : Inport  Port=2
  isBlueAlliance : Inport  Port=3
  Robot_Position_X : Inport  Port=4
  Robot_Velocity_X : Inport  Port=5
  Robot_Velocity_Y : Inport  Port=6
  Desired_Gyro_Angle : Inport  Port=7
  Gyro_Angle_Field_rad : Inport  Port=8
  Allowed_Shoot_Gyro_Error_rad : Inport  Port=9
  Desired_Shooter_Speed : Inport  Port=10
  Desired_Hood_Pos_Shoot : Inport  Port=11
  Estimated_Hood_Pos : Inport  Port=12
  Can_Pass : Inport  Port=13
  Measured_Shooter_Speed_Max : Inport  Port=14
  AND : Logic  Inputs=3  AllPortsSameDT=off  OutDataTypeStr=boolean
  AND{1..4} (4 alike) : Logic  AllPortsSameDT=off  OutDataTypeStr=boolean
  Abs : Abs  SaturateOnIntegerOverflow=off
  Abs1 : Abs  SaturateOnIntegerOverflow=off
  Abs4 : Abs  SaturateOnIntegerOverflow=off
  Angle Modulus : Controls_Components_lib/Angle Modulus  SystemSampleTime=-1  VariantActivationTime=update diagram  AllowFlexibleInterface=on  Latency=0  AutoFrameSizeCalculation=off
  Check if allowed to score in alliance zone : Subsystem
  Check if outside alliance zone : Subsystem
  Constant : Constant  Value=Rebuilt_Shoot_Robot_Velocity_Max
  Constant1 : Constant  Value=Rebuilt_Shoot_Hood_Pos_Max_Error
  Constant2 : Constant  Value=Rebuilt_Shoot_Motor_Max_Error
  GreaterThan : RelationalOperator  Operator=<=  OutDataTypeStr=boolean  RndMeth=Simplest  InputSameDT=off
  Hypot : Math  Operator=hypot
  OR : Logic  Operator=OR  AllPortsSameDT=off  OutDataTypeStr=boolean
  Relational Operator : RelationalOperator  Operator=<=  OutDataTypeStr=boolean  RndMeth=Simplest  InputSameDT=off
  Relational Operator1 : RelationalOperator  Operator=<=  OutDataTypeStr=boolean  RndMeth=Simplest  InputSameDT=off
  Relational Operator4 : RelationalOperator  Operator=<=  OutDataTypeStr=boolean  RndMeth=Simplest  InputSameDT=off
  Signal Copy : SignalConversion  OverrideOpt=off
  Subtract : Sum  Inputs=+-
  Subtract1 : Sum  Inputs=+-
  Subtract4 : Sum  Inputs=+-
  Ready_to_Score : Outport
  Ready_to_Pass : Outport  Port=2
  Ready_to_Unload_Manual : Outport  Port=3
  Is_Outside_Alliance_Zone : Outport  Port=4
  wires:
  Can_Pass/1 -> OR/2
  OR/1 -> AND/1
  AND4/1 -> Ready_to_Unload_Manual/1
  Angle Modulus/1 -> Abs/1
  Signal Copy/1 -> AND3/1  "RB_Logic_Outside_Zone"
  Estimated_Hood_Pos/1 -> Subtract4/2
  Relational Operator4/1 -> AND4/2, AND/3  "RB_Logic_Hood_Pos"
  Measured_Shooter_Speed_Max/1 -> Subtract1/2
  Hypot/1 -> GreaterThan/1
  Robot_Velocity_Y/1 -> Hypot/2
  Robot_Velocity_X/1 -> Hypot/1
  AND3/1 -> Ready_to_Pass/1  "RB_Ready_to_Pass"
  Check if outside alliance zone/1(Is_Outside_Alliance_Zone) -> Is_Outside_Alliance_Zone/1, Signal Copy/1
  AND2/1 -> Ready_to_Score/1  "RB_Ready_to_Score"
  AND/1 -> AND3/2, AND2/2
  AND1/1 -> AND2/1
  GreaterThan/1 -> AND1/2  "RB_Logic_Velocity"
  Check if allowed to score in alliance zone/1(Allow_Score_In_Alliance_Zone) -> AND1/1
  Constant1/1 -> Relational Operator4/2
  Abs4/1 -> Relational Operator4/1
  Subtract4/1 -> Abs4/1
  Allowed_Shoot_Gyro_Error_rad/1 -> Relational Operator/2
  Desired_Shooter_Speed/1 -> Subtract1/1
  Desired_Gyro_Angle/1 -> Subtract/1
  Gyro_Angle_Field_rad/1 -> Subtract/2
  Desired_Hood_Pos_Shoot/1 -> Subtract4/1
  Subtract1/1 -> Abs1/1
  Abs1/1 -> Relational Operator1/1
  Constant2/1 -> Relational Operator1/2
  Relational Operator1/1 -> AND4/1, AND/2  "RB_Logic_Shooter_Speed"
  Relational Operator/1 -> OR/1  "RB_Logic_Gyro_Angle"
  Abs/1 -> Relational Operator/1
  Subtract/1 -> Angle Modulus/1
  isRedHubActive/1 -> Check if allowed to score in alliance zone/3(isRedHubActive)
  isBlueAlliance/1 -> Check if allowed to score in alliance zone/1(isBlueAlliance), Check if outside alliance zone/1(isBlueAlliance)
  isBlueHubActive/1 -> Check if allowed to score in alliance zone/2(isBlueHubActive)
  Robot_Position_X/1 -> Check if allowed to score in alliance zone/4(Robot_Position_X), Check if outside alliance zone/2(Robot_Position_X)
  Constant/1 -> GreaterThan/2

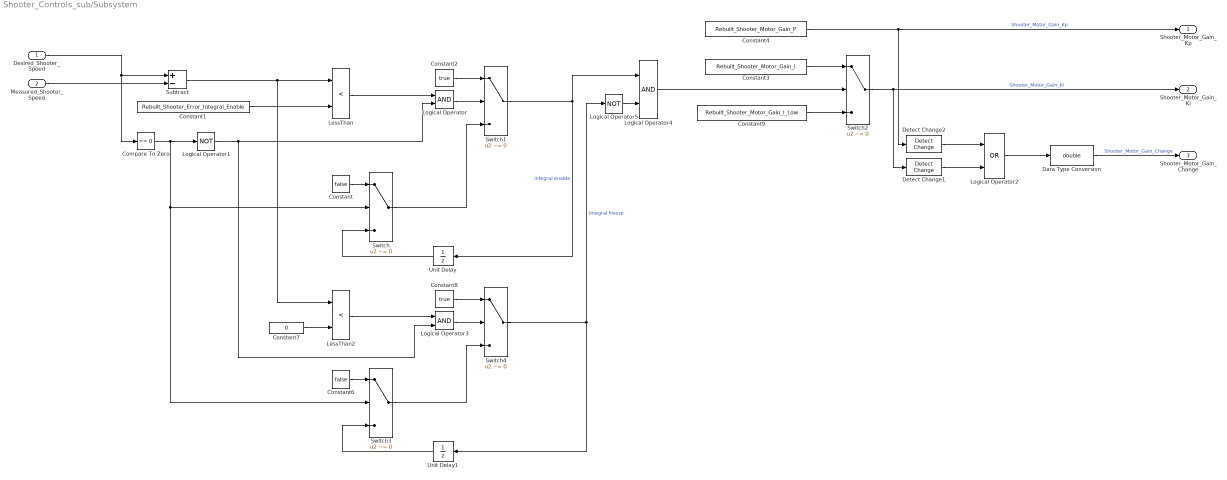
== system Shooter_Controls_sub/Subsystem ==
  Desired_Shooter_Speed : Inport
  Measured_Shooter_Speed : Inport  Port=2
  Compare To Zero : simulink/Logic and Bit Operations/Compare To Zero  relop===  OutDataTypeStr=boolean
  Constant : Constant  Value=false
  Constant1 : Constant  Value=Rebuilt_Shooter_Error_Integral_Enable
  Constant2 : Constant  Value=true
  Constant3 : Constant  Value=Rebuilt_Shooter_Motor_Gain_I
  Constant4 : Constant  Value=Rebuilt_Shooter_Motor_Gain_P
  Constant6 : Constant  Value=false
  Constant7 : Constant  Value=0
  Constant8 : Constant  Value=true
  Constant9 : Constant  Value=Rebuilt_Shooter_Motor_Gain_I_Low
  Data Type Conversion : DataTypeConversion  OutDataTypeStr=double  SaturateOnIntegerOverflow=off  RndMeth=Floor
  Detect Change1 : simulink/Logic and Bit Operations/Detect Change  vinit=0  OutDataTypeStr=boolean
  Detect Change2 : simulink/Logic and Bit Operations/Detect Change  vinit=0  OutDataTypeStr=boolean
  LessThan : RelationalOperator  Operator=<  OutDataTypeStr=boolean  RndMeth=Simplest  InputSameDT=off
  LessThan2 : RelationalOperator  Operator=<  OutDataTypeStr=boolean  RndMeth=Simplest  InputSameDT=off
  Logical Operator : Logic  AllPortsSameDT=off  OutDataTypeStr=boolean
  Logical Operator1 : Logic  Operator=NOT  AllPortsSameDT=off  OutDataTypeStr=boolean
  Logical Operator2 : Logic  Operator=OR  AllPortsSameDT=off  OutDataTypeStr=boolean
  Logical Operator3 : Logic  AllPortsSameDT=off  OutDataTypeStr=boolean
  Logical Operator4 : Logic  AllPortsSameDT=off  OutDataTypeStr=boolean
  Logical Operator5 : Logic  Operator=NOT  AllPortsSameDT=off  OutDataTypeStr=boolean
  Subtract : Sum  Inputs=+-
  Switch{,1..4} (5 alike) : Switch  Criteria=u2 ~= 0  SaturateOnIntegerOverflow=off  InputSameDT=off
  Unit Delay : UnitDelay  SampleTime=-1  HasFrameUpgradeWarning=on
  Unit Delay1 : UnitDelay  SampleTime=-1  HasFrameUpgradeWarning=on
  Shooter_Motor_Gain_Kp : Outport
  Shooter_Motor_Gain_Ki : Outport  Port=2
  Shooter_Motor_Gain_Change : Outport  Port=3
  wires:
  Constant9/1 -> Switch2/3
  Logical Operator4/1 -> Switch2/2
  Logical Operator5/1 -> Logical Operator4/2
  Constant6/1 -> Switch3/1
  Logical Operator3/1 -> Switch4/2
  Unit Delay1/1 -> Switch3/3
  LessThan2/1 -> Logical Operator3/1
  Compare To Zero/1 -> Logical Operator1/1, Switch/2, Switch3/2
  Constant7/1 -> LessThan2/2
  Constant8/1 -> Switch4/1
  Logical Operator/1 -> Switch1/2
  Constant1/1 -> LessThan/2
  Desired_Shooter_Speed/1 -> Compare To Zero/1, Subtract/1
  Constant/1 -> Switch/1
  Logical Operator1/1 -> Logical Operator3/2, Logical Operator/2
  Switch4/1 -> Logical Operator5/1, Unit Delay1/1  "integral freeze"
  Measured_Shooter_Speed/1 -> Subtract/2
  Switch3/1 -> Switch4/3
  Subtract/1 -> LessThan/1, LessThan2/1
  Switch/1 -> Switch1/3
  LessThan/1 -> Logical Operator/1
  Unit Delay/1 -> Switch/3
  Switch1/1 -> Unit Delay/1, Logical Operator4/1  "integral enable"
  Constant2/1 -> Switch1/1
  Constant3/1 -> Switch2/1
  Data Type Conversion/1 -> Shooter_Motor_Gain_Change/1  "Shooter_Motor_Gain_Change"
  Detect Change2/1 -> Logical Operator2/1
  Detect Change1/1 -> Logical Operator2/2
  Logical Operator2/1 -> Data Type Conversion/1
  Constant4/1 -> Shooter_Motor_Gain_Kp/1, Detect Change2/1  "Shooter_Motor_Gain_Kp"
  Switch2/1 -> Shooter_Motor_Gain_Ki/1, Detect Change1/1  "Shooter_Motor_Gain_Ki"

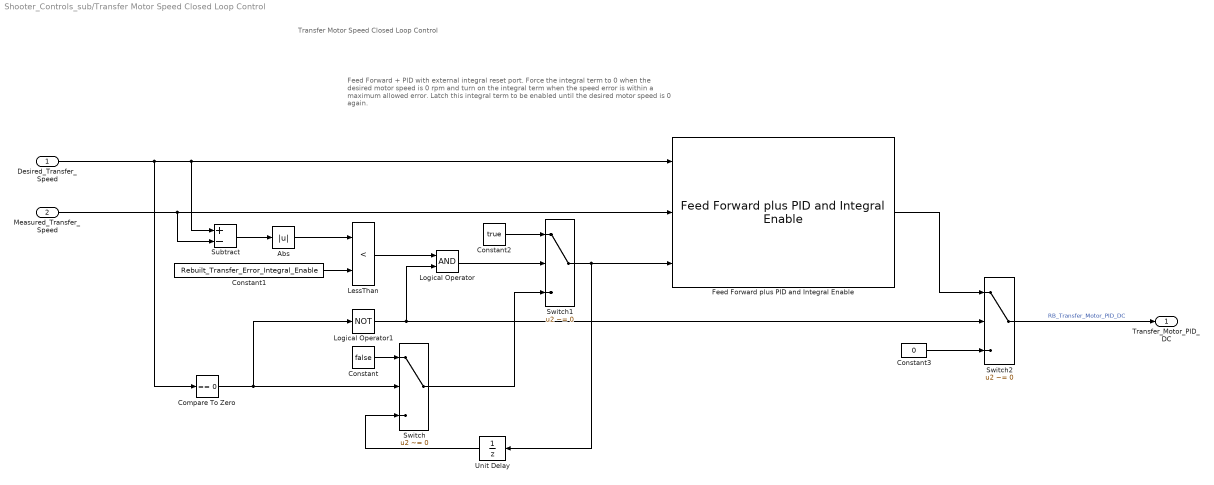
== system Shooter_Controls_sub/Transfer Motor Speed Closed Loop Control ==
  note: Transfer Motor Speed Closed Loop Control
  note: Feed Forward + PID with external integral reset port.
      |
      | Force the integral term to 0 when the desired motor speed is 0 rpm and turn on the integral term when the speed error is within a maximum allowed error.  Latch this integral term to be enabled until the desired motor speed is 0 again.
  Desired_Transfer_Speed : Inport
  Measured_Transfer_Speed : Inport  Port=2
  Abs : Abs  SaturateOnIntegerOverflow=off
  Compare To Zero : simulink/Logic and Bit Operations/Compare To Zero  relop===  OutDataTypeStr=boolean
  Constant : Constant  Value=false
  Constant1 : Constant  Value=Rebuilt_Transfer_Error_Integral_Enable
  Constant2 : Constant  Value=true
  Constant3 : Constant  Value=0
  Feed Forward plus PID and Integral Enable : Controls_Components_lib/Feed Forward plus PID and Integral Enable  Gain_FF=Rebuilt_Transfer_Motor_Gain_FF  Gain_P=Rebuilt_Transfer_Motor_Gain_P  Gain_I=Rebuilt_Transfer_Motor_Gain_I  Gain_D=0  FilterCoeff_D=0.1  Limit_I_Upper=0.1  Limit_I_Lower=-0.1  Limit_D_Upper=0.1  Limit_D_Lower=-0.1  Limit_T_Upper=1  Limit_T_Lower=-1
  LessThan : RelationalOperator  Operator=<  OutDataTypeStr=boolean  RndMeth=Simplest  InputSameDT=off
  Logical Operator : Logic  AllPortsSameDT=off  OutDataTypeStr=boolean
  Logical Operator1 : Logic  Operator=NOT  AllPortsSameDT=off  OutDataTypeStr=boolean
  Subtract : Sum  Inputs=+-
  Switch : Switch  Criteria=u2 ~= 0  SaturateOnIntegerOverflow=off  InputSameDT=off
  Switch1 : Switch  Criteria=u2 ~= 0  SaturateOnIntegerOverflow=off  InputSameDT=off
  Switch2 : Switch  Criteria=u2 ~= 0  SaturateOnIntegerOverflow=off  InputSameDT=off
  Unit Delay : UnitDelay  SampleTime=-1  HasFrameUpgradeWarning=on
  Transfer_Motor_PID_DC : Outport
  wires:
  Feed Forward plus PID and Integral Enable/1 -> Switch2/1
  Switch2/1 -> Transfer_Motor_PID_DC/1  "RB_Transfer_Motor_PID_DC"
  Constant3/1 -> Switch2/3
  Unit Delay/1 -> Switch/3
  Switch/1 -> Switch1/3
  Switch1/1 -> Feed Forward plus PID and Integral Enable/3, Unit Delay/1
  Constant2/1 -> Switch1/1
  Constant/1 -> Switch/1
  Compare To Zero/1 -> Logical Operator1/1, Switch/2
  Desired_Transfer_Speed/1 -> Subtract/1, Feed Forward plus PID and Integral Enable/1, Compare To Zero/1
  Measured_Transfer_Speed/1 -> Feed Forward plus PID and Integral Enable/2, Subtract/2
  Abs/1 -> LessThan/1
  Constant1/1 -> LessThan/2
  Subtract/1 -> Abs/1
  LessThan/1 -> Logical Operator/1
  Logical Operator/1 -> Switch1/2
  Logical Operator1/1 -> Switch2/2, Logical Operator/2

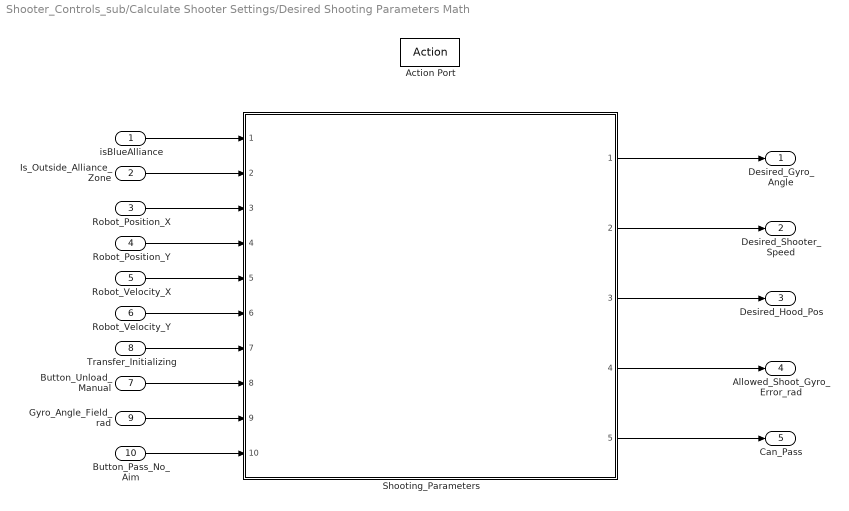
== system Shooter_Controls_sub/Calculate Shooter Settings/Desired Shooting Parameters Math ==
  isBlueAlliance : Inport
  Is_Outside_Alliance_Zone : Inport  Port=2
  Robot_Position_X : Inport  Port=3
  Robot_Position_Y : Inport  Port=4
  Robot_Velocity_X : Inport  Port=5
  Robot_Velocity_Y : Inport  Port=6
  Button_Unload_Manual : Inport  Port=7
  Transfer_Initializing : Inport  Port=8
  Gyro_Angle_Field_rad : Inport  Port=9
  Button_Pass_No_Aim : Inport  Port=10
  Action Port : ActionPort
  Shooting_Parameters : Subsystem  ReferencedSubsystem=Shooting_Parameters_sub
  Desired_Gyro_Angle : Outport
  Desired_Shooter_Speed : Outport  Port=2
  Desired_Hood_Pos : Outport  Port=3
  Allowed_Shoot_Gyro_Error_rad : Outport  Port=4
  Can_Pass : Outport  Port=5
  wires:
  Shooting_Parameters/5 -> Can_Pass/1
  Button_Pass_No_Aim/1 -> Shooting_Parameters/10
  Gyro_Angle_Field_rad/1 -> Shooting_Parameters/9
  Button_Unload_Manual/1 -> Shooting_Parameters/8
  Transfer_Initializing/1 -> Shooting_Parameters/7
  Is_Outside_Alliance_Zone/1 -> Shooting_Parameters/2
  Shooting_Parameters/4 -> Allowed_Shoot_Gyro_Error_rad/1
  Shooting_Parameters/3 -> Desired_Hood_Pos/1
  Shooting_Parameters/2 -> Desired_Shooter_Speed/1
  Shooting_Parameters/1 -> Desired_Gyro_Angle/1
  Robot_Velocity_Y/1 -> Shooting_Parameters/6
  Robot_Velocity_X/1 -> Shooting_Parameters/5
  Robot_Position_Y/1 -> Shooting_Parameters/4
  Robot_Position_X/1 -> Shooting_Parameters/3
  isBlueAlliance/1 -> Shooting_Parameters/1

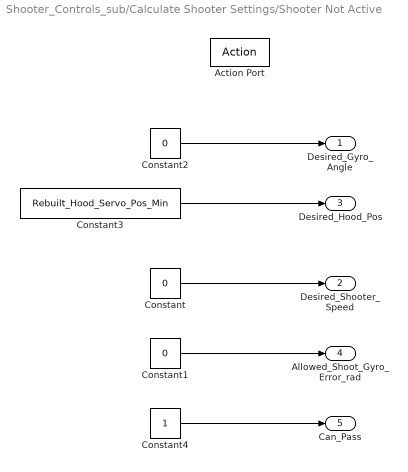
== system Shooter_Controls_sub/Calculate Shooter Settings/Shooter Not Active ==
  Action Port : ActionPort
  Constant : Constant  Value=0
  Constant1 : Constant  Value=0
  Constant2 : Constant  Value=0
  Constant3 : Constant  Value=Rebuilt_Hood_Servo_Pos_Min
  Constant4 : Constant  OutDataTypeStr=boolean
  Desired_Gyro_Angle : Outport
  Desired_Shooter_Speed : Outport  Port=2
  Desired_Hood_Pos : Outport  Port=3
  Allowed_Shoot_Gyro_Error_rad : Outport  Port=4
  Can_Pass : Outport  Port=5
  wires:
  Constant4/1 -> Can_Pass/1
  Constant3/1 -> Desired_Hood_Pos/1
  Constant2/1 -> Desired_Gyro_Angle/1
  Constant1/1 -> Allowed_Shoot_Gyro_Error_rad/1
  Constant/1 -> Desired_Shooter_Speed/1

== system Shooter_Controls_sub/Check if Hub is Active for Scoring/If Action Subsystem ==
  Action Port : ActionPort  InitializeStates=reset
  Constant : Constant  OutDataTypeStr=boolean
  Constant1 : Constant  Value=0.020
  Signal Copy : SignalConversion  OverrideOpt=off
  Sum : Sum  Inputs=|-+
  Unit Delay : UnitDelay  InitialCondition=Rebuilt_Match_Time_Auto_Timer  SampleTime=-1  HasFrameUpgradeWarning=on
      settings: AttributesFormatString=Initial Condition = %<InitialCondition>
  IsBlueActive : Outport
  IsRedActive : Outport  Port=2
  Time_Remaining : Outport  Port=3
  wires:
  Signal Copy/1 -> Time_Remaining/1
  Unit Delay/1 -> Sum/2
  Sum/1 -> Signal Copy/1, Unit Delay/1
  Constant1/1 -> Sum/1
  Constant/1 -> IsBlueActive/1, IsRedActive/1

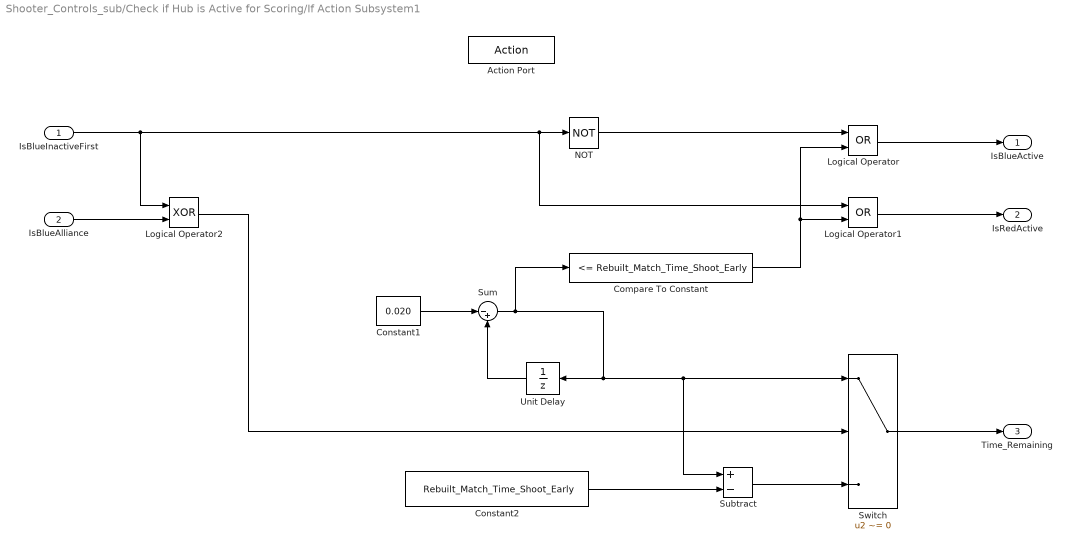
== system Shooter_Controls_sub/Check if Hub is Active for Scoring/If Action Subsystem1 ==
  IsBlueInactiveFirst : Inport
  IsBlueAlliance : Inport  Port=2
  Action Port : ActionPort  InitializeStates=reset
  Compare To Constant : simulink/Logic and Bit Operations/Compare To Constant  relop=<=  const=Rebuilt_Match_Time_Shoot_Early  OutDataTypeStr=boolean
  Constant1 : Constant  Value=0.020
  Constant2 : Constant  Value=Rebuilt_Match_Time_Shoot_Early
  Logical Operator : Logic  Operator=OR  AllPortsSameDT=off  OutDataTypeStr=boolean
  Logical Operator1 : Logic  Operator=OR  AllPortsSameDT=off  OutDataTypeStr=boolean
  Logical Operator2 : Logic  Operator=XOR  AllPortsSameDT=off  OutDataTypeStr=boolean
  NOT : Logic  Operator=NOT  AllPortsSameDT=off  OutDataTypeStr=boolean
  Subtract : Sum  Inputs=+-
  Sum : Sum  Inputs=|-+
  Switch : Switch  Criteria=u2 ~= 0  SaturateOnIntegerOverflow=off  InputSameDT=off
  Unit Delay : UnitDelay  InitialCondition=Rebuilt_Match_Time_Shift_Timer  SampleTime=-1  HasFrameUpgradeWarning=on
      settings: AttributesFormatString=Initial Condition = %<InitialCondition>
  IsBlueActive : Outport
  IsRedActive : Outport  Port=2
  Time_Remaining : Outport  Port=3
  wires:
  Constant2/1 -> Subtract/2
  Subtract/1 -> Switch/3
  Switch/1 -> Time_Remaining/1
  Logical Operator2/1 -> Switch/2
  IsBlueAlliance/1 -> Logical Operator2/2
  Logical Operator1/1 -> IsRedActive/1
  Compare To Constant/1 -> Logical Operator/2, Logical Operator1/2
  Logical Operator/1 -> IsBlueActive/1
  NOT/1 -> Logical Operator/1
  Sum/1 -> Unit Delay/1, Switch/1, Subtract/1, Compare To Constant/1
  Unit Delay/1 -> Sum/2
  Constant1/1 -> Sum/1
  IsBlueInactiveFirst/1 -> NOT/1, Logical Operator1/1, Logical Operator2/1

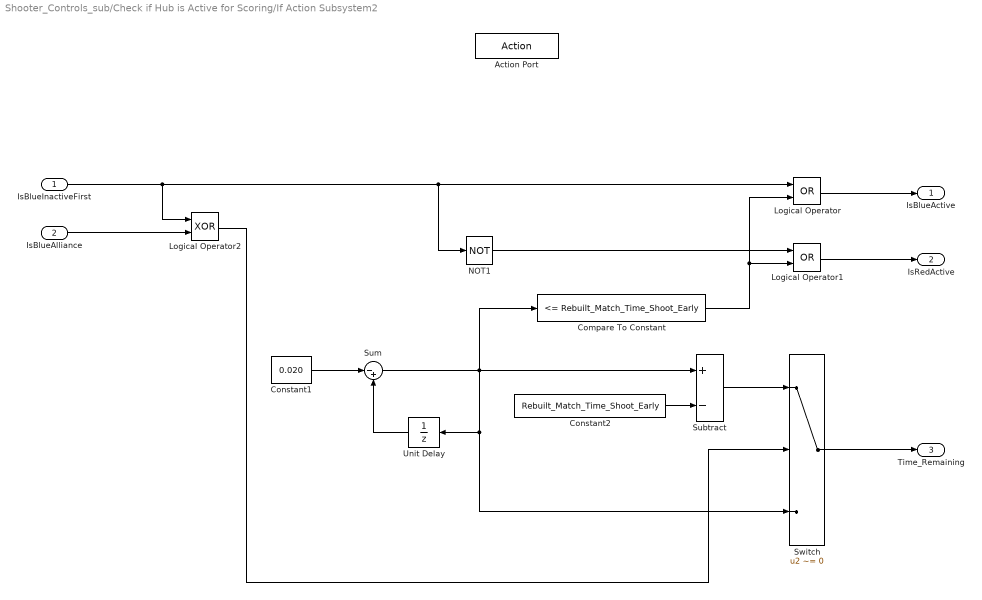
== system Shooter_Controls_sub/Check if Hub is Active for Scoring/If Action Subsystem2 ==
  IsBlueInactiveFirst : Inport
  IsBlueAlliance : Inport  Port=2
  Action Port : ActionPort  InitializeStates=reset
  Compare To Constant : simulink/Logic and Bit Operations/Compare To Constant  relop=<=  const=Rebuilt_Match_Time_Shoot_Early  OutDataTypeStr=boolean
  Constant1 : Constant  Value=0.020
  Constant2 : Constant  Value=Rebuilt_Match_Time_Shoot_Early
  Logical Operator : Logic  Operator=OR  AllPortsSameDT=off  OutDataTypeStr=boolean
  Logical Operator1 : Logic  Operator=OR  AllPortsSameDT=off  OutDataTypeStr=boolean
  Logical Operator2 : Logic  Operator=XOR  AllPortsSameDT=off  OutDataTypeStr=boolean
  NOT1 : Logic  Operator=NOT  AllPortsSameDT=off  OutDataTypeStr=boolean
  Subtract : Sum  Inputs=+-
  Sum : Sum  Inputs=|-+
  Switch : Switch  Criteria=u2 ~= 0  SaturateOnIntegerOverflow=off  InputSameDT=off
  Unit Delay : UnitDelay  InitialCondition=Rebuilt_Match_Time_Shift_Timer  SampleTime=-1  HasFrameUpgradeWarning=on
      settings: AttributesFormatString=Initial Condition = %<InitialCondition>
  IsBlueActive : Outport
  IsRedActive : Outport  Port=2
  Time_Remaining : Outport  Port=3
  wires:
  Constant2/1 -> Subtract/2
  Subtract/1 -> Switch/1
  Logical Operator2/1 -> Switch/2
  IsBlueAlliance/1 -> Logical Operator2/2
  Switch/1 -> Time_Remaining/1
  Logical Operator1/1 -> IsRedActive/1
  Logical Operator/1 -> IsBlueActive/1
  Compare To Constant/1 -> Logical Operator/2, Logical Operator1/2
  Sum/1 -> Compare To Constant/1, Subtract/1, Unit Delay/1, Switch/3
  Unit Delay/1 -> Sum/2
  Constant1/1 -> Sum/1
  NOT1/1 -> Logical Operator1/1
  IsBlueInactiveFirst/1 -> Logical Operator/1, NOT1/1, Logical Operator2/1

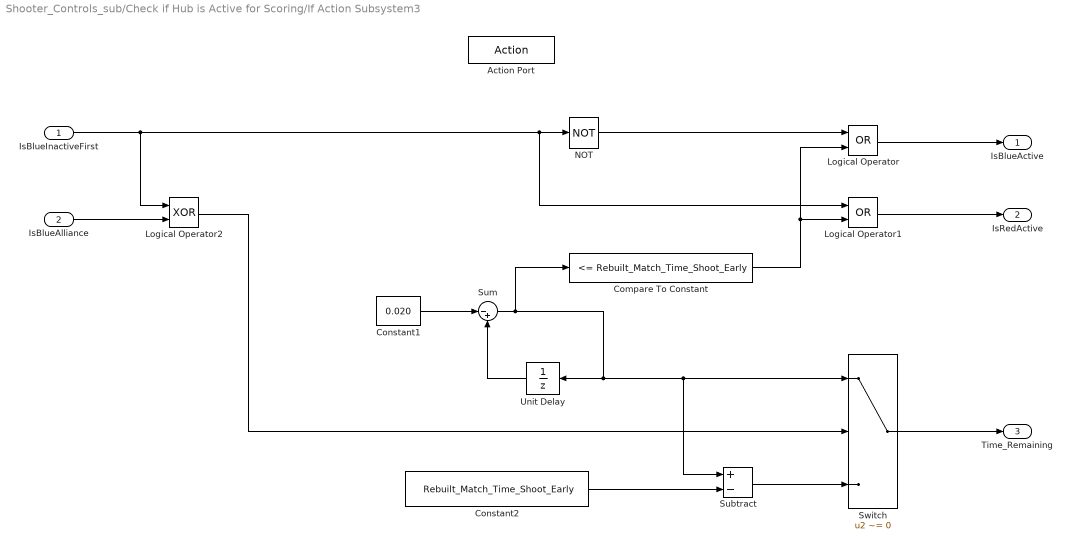
== system Shooter_Controls_sub/Check if Hub is Active for Scoring/If Action Subsystem3 ==
  IsBlueInactiveFirst : Inport
  IsBlueAlliance : Inport  Port=2
  Action Port : ActionPort  InitializeStates=reset
  Compare To Constant : simulink/Logic and Bit Operations/Compare To Constant  relop=<=  const=Rebuilt_Match_Time_Shoot_Early  OutDataTypeStr=boolean
  Constant1 : Constant  Value=0.020
  Constant2 : Constant  Value=Rebuilt_Match_Time_Shoot_Early
  Logical Operator : Logic  Operator=OR  AllPortsSameDT=off  OutDataTypeStr=boolean
  Logical Operator1 : Logic  Operator=OR  AllPortsSameDT=off  OutDataTypeStr=boolean
  Logical Operator2 : Logic  Operator=XOR  AllPortsSameDT=off  OutDataTypeStr=boolean
  NOT : Logic  Operator=NOT  AllPortsSameDT=off  OutDataTypeStr=boolean
  Subtract : Sum  Inputs=+-
  Sum : Sum  Inputs=|-+
  Switch : Switch  Criteria=u2 ~= 0  SaturateOnIntegerOverflow=off  InputSameDT=off
  Unit Delay : UnitDelay  InitialCondition=Rebuilt_Match_Time_Shift_Timer  SampleTime=-1  HasFrameUpgradeWarning=on
      settings: AttributesFormatString=Initial Condition = %<InitialCondition>
  IsBlueActive : Outport
  IsRedActive : Outport  Port=2
  Time_Remaining : Outport  Port=3
  wires:
  IsBlueInactiveFirst/1 -> Logical Operator2/1, Logical Operator1/1, NOT/1
  Constant1/1 -> Sum/1
  Unit Delay/1 -> Sum/2
  Sum/1 -> Compare To Constant/1, Subtract/1, Switch/1, Unit Delay/1
  NOT/1 -> Logical Operator/1
  Logical Operator/1 -> IsBlueActive/1
  Compare To Constant/1 -> Logical Operator1/2, Logical Operator/2
  Logical Operator1/1 -> IsRedActive/1
  IsBlueAlliance/1 -> Logical Operator2/2
  Logical Operator2/1 -> Switch/2
  Switch/1 -> Time_Remaining/1
  Subtract/1 -> Switch/3
  Constant2/1 -> Subtract/2

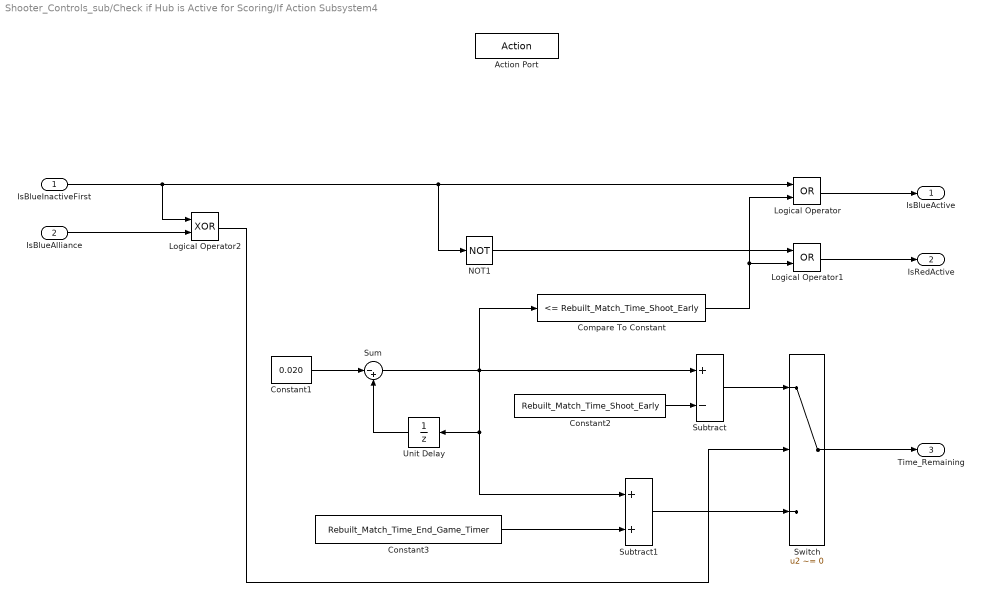
== system Shooter_Controls_sub/Check if Hub is Active for Scoring/If Action Subsystem4 ==
  IsBlueInactiveFirst : Inport
  IsBlueAlliance : Inport  Port=2
  Action Port : ActionPort  InitializeStates=reset
  Compare To Constant : simulink/Logic and Bit Operations/Compare To Constant  relop=<=  const=Rebuilt_Match_Time_Shoot_Early  OutDataTypeStr=boolean
  Constant1 : Constant  Value=0.020
  Constant2 : Constant  Value=Rebuilt_Match_Time_Shoot_Early
  Constant3 : Constant  Value=Rebuilt_Match_Time_End_Game_Timer
  Logical Operator : Logic  Operator=OR  AllPortsSameDT=off  OutDataTypeStr=boolean
  Logical Operator1 : Logic  Operator=OR  AllPortsSameDT=off  OutDataTypeStr=boolean
  Logical Operator2 : Logic  Operator=XOR  AllPortsSameDT=off  OutDataTypeStr=boolean
  NOT1 : Logic  Operator=NOT  AllPortsSameDT=off  OutDataTypeStr=boolean
  Subtract : Sum  Inputs=+-
  Subtract1 : Sum
  Sum : Sum  Inputs=|-+
  Switch : Switch  Criteria=u2 ~= 0  SaturateOnIntegerOverflow=off  InputSameDT=off
  Unit Delay : UnitDelay  InitialCondition=Rebuilt_Match_Time_Shift_Timer  SampleTime=-1  HasFrameUpgradeWarning=on
      settings: AttributesFormatString=Initial Condition = %<InitialCondition>
  IsBlueActive : Outport
  IsRedActive : Outport  Port=2
  Time_Remaining : Outport  Port=3
  wires:
  Constant3/1 -> Subtract1/2
  Subtract1/1 -> Switch/3
  IsBlueInactiveFirst/1 -> Logical Operator2/1, NOT1/1, Logical Operator/1
  NOT1/1 -> Logical Operator1/1
  Constant1/1 -> Sum/1
  Unit Delay/1 -> Sum/2
  Sum/1 -> Unit Delay/1, Subtract1/1, Subtract/1, Compare To Constant/1
  Compare To Constant/1 -> Logical Operator1/2, Logical Operator/2
  Logical Operator/1 -> IsBlueActive/1
  Logical Operator1/1 -> IsRedActive/1
  Switch/1 -> Time_Remaining/1
  IsBlueAlliance/1 -> Logical Operator2/2
  Logical Operator2/1 -> Switch/2
  Subtract/1 -> Switch/1
  Constant2/1 -> Subtract/2

== system Shooter_Controls_sub/Check if Hub is Active for Scoring/If Action Subsystem5 ==
  Action Port : ActionPort  InitializeStates=reset
  Constant : Constant  OutDataTypeStr=boolean
  Constant1 : Constant  Value=0.020
  Signal Copy : SignalConversion  OverrideOpt=off
  Sum : Sum  Inputs=|-+
  Unit Delay : UnitDelay  InitialCondition=Rebuilt_Match_Time_End_Game_Timer  SampleTime=-1  HasFrameUpgradeWarning=on
      settings: AttributesFormatString=Initial Condition = %<InitialCondition>
  IsBlueActive : Outport
  IsRedActive : Outport  Port=2
  Time_Remaining : Outport  Port=3
  wires:
  Sum/1 -> Signal Copy/1, Unit Delay/1
  Unit Delay/1 -> Sum/2
  Signal Copy/1 -> Time_Remaining/1
  Constant1/1 -> Sum/1
  Constant/1 -> IsRedActive/1, IsBlueActive/1

== system Shooter_Controls_sub/Check if Hub is Active for Scoring/Subsystem ==
  Reset : Inport
  Constant : Constant  Value=0
  Constant4 : Constant  Value=t_sample
  Sum : Sum  Inputs=|++
  Switch : Switch  Criteria=u2 ~= 0  SaturateOnIntegerOverflow=off  InputSameDT=off
  Unit Delay : UnitDelay  SampleTime=-1  HasFrameUpgradeWarning=on
  Time : Outport
  wires:
  Unit Delay/1 -> Switch/3
  Switch/1 -> Sum/2
  Constant/1 -> Switch/1
  Reset/1 -> Switch/2
  Sum/1 -> Time/1, Unit Delay/1
  Constant4/1 -> Sum/1

== system Shooter_Controls_sub/Check if Hub is Active for Scoring/Subsystem1 ==
  Reset : Inport
  Constant : Constant  Value=0
  Constant4 : Constant  Value=t_sample
  Sum : Sum  Inputs=|++
  Switch : Switch  Criteria=u2 ~= 0  SaturateOnIntegerOverflow=off  InputSameDT=off
  Unit Delay : UnitDelay  SampleTime=-1  HasFrameUpgradeWarning=on
  Time : Outport
  wires:
  Constant4/1 -> Sum/1
  Sum/1 -> Unit Delay/1, Time/1
  Reset/1 -> Switch/2
  Constant/1 -> Switch/1
  Switch/1 -> Sum/2
  Unit Delay/1 -> Switch/3

== system Shooter_Controls_sub/Ready_to_Shoot/Check if allowed to score in alliance zone ==
  note: Allow Score in Alliance Zone
  note: If we are blue alliance and the blue hub is active and the robot is in the blue alliance zone then allow shooting.
      |
      | If we are red alliance and the red hub is active and the robot is in the red alliance zone then allow shooting.
  isBlueAlliance : Inport
  isBlueHubActive : Inport  Port=2
  isRedHubActive : Inport  Port=3
  Robot_Position_X : Inport  Port=4
  Blue : Subsystem  TreatAsAtomicUnit=on
  If : If  IfExpression=u1 ~= 0
  Merge : Merge
  Red : Subsystem  TreatAsAtomicUnit=on
  Allow_Score_In_Alliance_Zone : Outport
  wires:
  If/2 -> Red/Action
  If/1 -> Blue/Action
  Merge/1 -> Allow_Score_In_Alliance_Zone/1  "RB_Logic_Score_In_Zone"
  Robot_Position_X/1 -> Red/2(Robot_Position_X), Blue/2(Robot_Position_X)
  isRedHubActive/1 -> Red/1(isRedHubActive)
  isBlueAlliance/1 -> If/1
  Blue/1(CanShootBlue) -> Merge/1
  isBlueHubActive/1 -> Blue/1(isBlueHubActive)
  Red/1(CanShootRed) -> Merge/2

== system Shooter_Controls_sub/Ready_to_Shoot/Check if outside alliance zone ==
  note: If we are blue alliance and the robot is outside the blue alliance zone then allow passing.
      |
      | If we are red alliance and the robot is outside the red alliance zone then allow passing.
  note: Allow Passing When Outside Our Alliance
  isBlueAlliance : Inport
  Robot_Position_X : Inport  Port=2
  Blue : Subsystem  TreatAsAtomicUnit=on
  If : If  IfExpression=u1 ~= 0
  Merge : Merge
  Red : Subsystem  TreatAsAtomicUnit=on
  Is_Outside_Alliance_Zone : Outport
  wires:
  If/2 -> Red/Action
  If/1 -> Blue/Action
  Merge/1 -> Is_Outside_Alliance_Zone/1  "Is_Outside_Alliance_Zone"
  Robot_Position_X/1 -> Red/1(Robot_Position_X), Blue/1(Robot_Position_X1)
  isBlueAlliance/1 -> If/1
  Blue/1(Can_Pass_Blue) -> Merge/1
  Red/1(Can_Pass_Red) -> Merge/2
